simulink library "suspended_payload_lib"  (R2018b)
settings: Solver=VariableStepAuto  StartTime=0.0  StopTime=10.0  RelTol=1e-3
undefined symbols (not defined in the file or in its folder): IC_susp_payload, susp_payload, uav
libraries: axes_transformation_lib x10, flight_parameters_lib x9, unit_conversions_lib x3, vrlib x2, rigidBody_lib x1
settings Model: Creator=jonas  LastModifiedBy=yannic

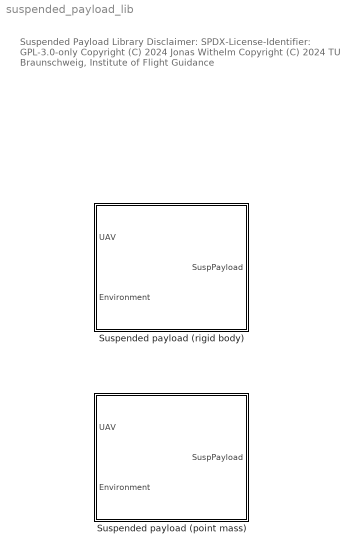
== system suspended_payload_lib ==
  note: Suspended Payload Library
      |
      | Disclaimer:
      | SPDX-License-Identifier: GPL-3.0-only
      |
      | Copyright (C) 2024 Jonas Withelm
      | Copyright (C) 2024 TU Braunschweig, Institute of Flight Guidance
  Suspended payload (point mass) : Subsystem  mask(Suspended payload (point mass)){uav_=uav, susp_payload_=susp_payload, IC_sp_=IC_susp_payload}
      mask prompts: uav_ "uav parameters struct"; susp_payload_ "suspended payload parameters struct"; IC_sp_ "suspended payload initial conditions struct"
      mask help: Point mass suspended payload model (without aerodynamics and joint angle limit)
  Suspended payload (rigid body) : Subsystem  mask(Suspended payload (rigid body)){uav_=uav, susp_payload_=susp_payload, IC_sp_=IC_susp_payload}
      mask prompts: uav_ "uav parameters struct"; susp_payload_ "suspended payload parameters struct"; IC_sp_ "suspended payload initial conditions struct"
      mask help: Rigid body suspended payload model with simple aerodynamics and joint angle limit

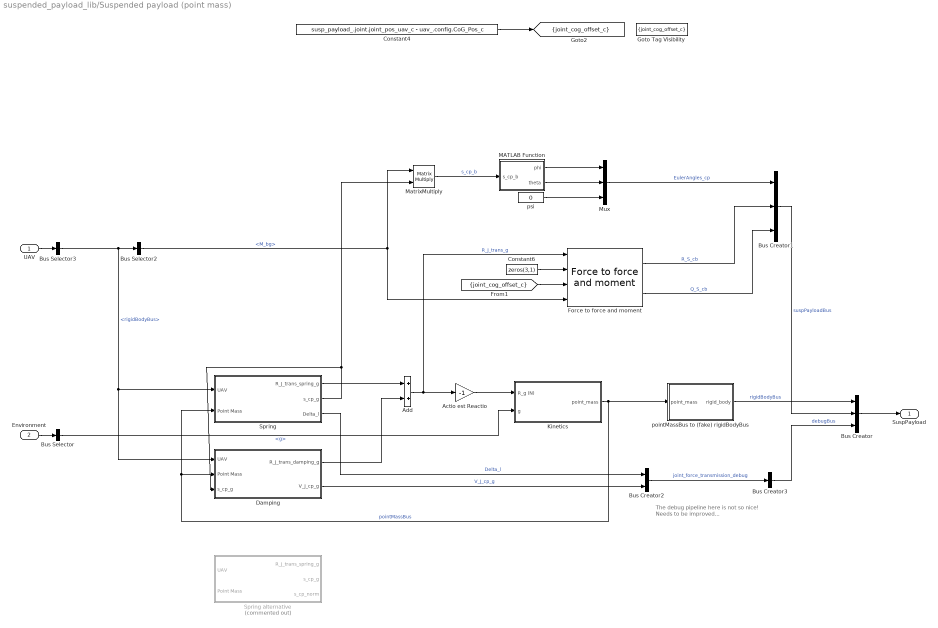
== system suspended_payload_lib/Suspended payload (point mass) ==
  note: The debug pipeline here is not so nice!
      |
      | Needs to be improved...
  UAV : Inport
  Environment : Inport  Port=2
  Actio est Reactio : Gain  Gain=-1
  Add : Sum
  Bus Creator : BusCreator  Inputs=3
  Bus Creator1 : BusCreator  Inputs=3
  Bus Creator2 : BusCreator  Inputs=2
  Bus Creator3 : BusCreator  Inputs=1
  Bus Selector : BusSelector  OutputSignals=g
  Bus Selector2 : BusSelector  OutputSignals=M_bg
  Bus Selector3 : BusSelector  OutputSignals=rigidBodyBus
  Constant4 : Constant  Value=susp_payload_.joint.joint_pos_uav_c - uav_.config.CoG_Pos_c
  Constant6 : Constant  Value=zeros(3,1)
  Damping : Subsystem
  Force to force and moment : axes_transformation_lib/Force to force and moment  SystemSampleTime=-1
      settings: SourceProductName=LADAC
  Goto Tag Visibility : GotoTagVisibility  GotoTag=joint_cog_offset_c
  Kinetics : Subsystem
  MATLAB Function : MATLAB Function  TreatAsAtomicUnit=on
  MatrixMultiply : Product  Multiplication=Matrix(*)
  Mux : Mux  Inputs=3
  Spring : Subsystem
  Spring alternative : Subsystem  Commented=on
  pointMassBus to (fake) rigidBodyBus : Subsystem
  psi : Constant  Value=0
  SuspPayload : Outport
  tag scope: joint_cog_offset_c=scoped
  wires:
  MATLAB Function/1(phi) -> Mux/1
  Constant6/1 -> Force to force and moment/2
  Spring/1(R_J_trans_spring_g) -> Add/1
  [joint_cog_offset_c] -> Force to force and moment/3
  Add/1 -> Force to force and moment/1, Actio est Reactio/1  "R_J_trans_g"
  MATLAB Function/2(theta) -> Mux/2
  MatrixMultiply/1 -> MATLAB Function/1(s_cp_b)  "s_cp_b"
  Bus Creator1/1 -> Bus Creator/2  "suspPayloadBus"
  Force to force and moment/1 -> Bus Creator1/2  "R_S_cb"
  Force to force and moment/2 -> Bus Creator1/3  "Q_S_cb"
  Bus Selector2/1 -> Force to force and moment/4, MatrixMultiply/1  "<M_bg>"
  UAV/1 -> Bus Selector3/1
  Spring/2(s_cp_g) -> MatrixMultiply/2, Damping/3(s_cp_g)
  Damping/1(R_J_trans_damping_g) -> Add/2
  Bus Creator/1 -> SuspPayload/1
  Kinetics/1(point_mass) -> Spring/2(Point Mass), Damping/2(Point Mass), pointMassBus to (fake) rigidBodyBus/1(point_mass)  "pointMassBus"
  pointMassBus to (fake) rigidBodyBus/1(rigid_body) -> Bus Creator/1  "rigidBodyBus"
  Actio est Reactio/1 -> Kinetics/1(R_g (N))
  Spring/3(Delta_l) -> Bus Creator2/1  "Delta_l"
  psi/1 -> Mux/3
  Environment/1 -> Bus Selector/1
  Damping/2(V_J_cp_g) -> Bus Creator2/2  "V_J_cp_g"
  Bus Creator2/1 -> Bus Creator3/1  "joint_force_transmission_debug"
  Bus Creator3/1 -> Bus Creator/3  "debugBus"
  Mux/1 -> Bus Creator1/1  "EulerAngles_cp"
  Bus Selector3/1 -> Spring/1(UAV), Damping/1(UAV), Bus Selector2/1  "<rigidBodyBus>"
  Constant4/1 -> [joint_cog_offset_c]
  Bus Selector/1 -> Kinetics/2(g)  "<g>"

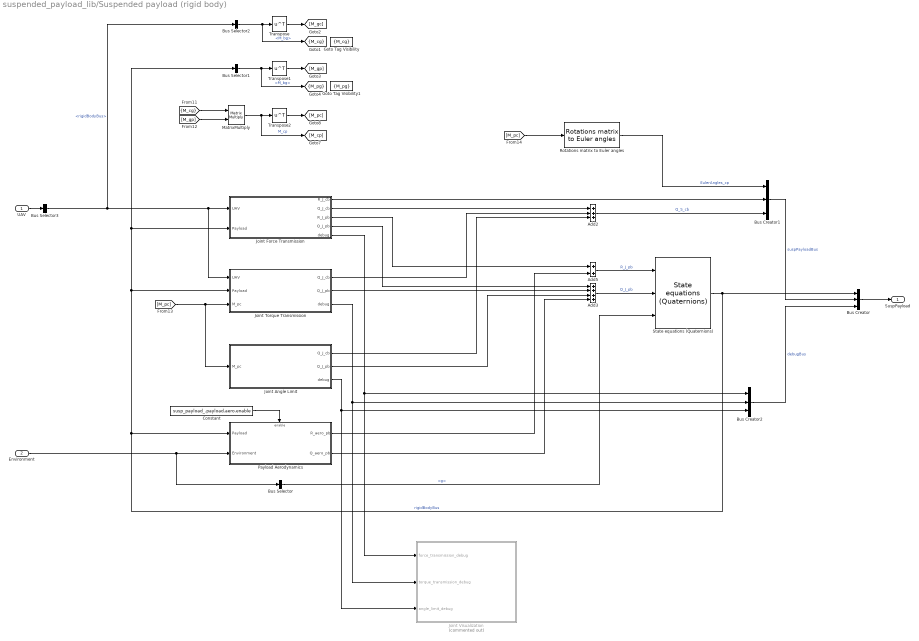
== system suspended_payload_lib/Suspended payload (rigid body) ==
  UAV : Inport
  Environment : Inport  Port=2
  Add2 : Sum  Inputs=+++
  Add3 : Sum  Inputs=++++
  Add5 : Sum
  Bus Creator : BusCreator  Inputs=3
  Bus Creator1 : BusCreator  Inputs=3
  Bus Creator2 : BusCreator  Inputs=3
  Bus Selector : BusSelector  OutputSignals=g
  Bus Selector1 : BusSelector  OutputSignals=M_bg
  Bus Selector2 : BusSelector  OutputSignals=M_bg
  Bus Selector3 : BusSelector  OutputSignals=rigidBodyBus
  Constant : Constant  Value=susp_payload_.payload.aero.enable
  Goto Tag Visibility : GotoTagVisibility  GotoTag=M_cg
  Goto Tag Visibility1 : GotoTagVisibility  GotoTag=M_pg
  Joint Angle Limit : Subsystem
  Joint Force Transmission : Subsystem
  Joint Torque Transmission : Subsystem
  Joint Visualization : Subsystem  Commented=on
  MatrixMultiply : Product  Multiplication=Matrix(*)
  Payload Aerodynamics : Subsystem
  Rotations matrix to Euler angles : axes_transformation_lib/Rotations matrix to Euler angles  SystemSampleTime=-1
      settings: SourceProductName=LADAC
  State equations (Quaternions) : rigidBody_lib/State equations (Quaternions)  m=susp_payload_.body.m  I=susp_payload_.body.I  is_g_checked=on  g=10  omega_Kb_0=IC_sp_.omega_Kb  q_bg_0=IC_sp_.q_bg  V_Kb_0=IC_sp_.V_Kb  s_g_0=IC_sp_.s_g
      settings: SourceProductName=LADAC
  Transpose : Math  Operator=transpose  SaturateOnIntegerOverflow=on
  Transpose1 : Math  Operator=transpose  SaturateOnIntegerOverflow=on
  Transpose2 : Math  Operator=transpose  SaturateOnIntegerOverflow=on
  SuspPayload : Outport
  tag scope: M_cg=scoped, M_pg=scoped
  wires:
  Bus Creator1/1 -> Bus Creator/2  "suspPayloadBus"
  Bus Selector/1 -> State equations (Quaternions)/3  "<g>"
  Add2/1 -> Bus Creator1/3  "Q_S_cb"
  MatrixMultiply/1 -> [M_cp], Transpose2/1  "M_cp"
  [M_gp] -> MatrixMultiply/2
  [M_cg] -> MatrixMultiply/1
  [M_pc] -> Joint Angle Limit/1(M_pc), Joint Torque Transmission/3(M_pc)
  [M_pc] -> Rotations matrix to Euler angles/1
  Transpose2/1 -> [M_pc]
  Add3/1 -> State equations (Quaternions)/2  "Q_J_pb"
  Joint Angle Limit/1(Q_J_cb) -> Add2/3
  Joint Angle Limit/2(Q_J_pb) -> Add3/3
  Joint Torque Transmission/1(Q_J_cb) -> Add2/2
  Joint Torque Transmission/2(Q_J_pb) -> Add3/2
  Environment/1 -> Bus Selector/1, Payload Aerodynamics/2(Environment)
  Add5/1 -> State equations (Quaternions)/1  "R_J_pb"
  Payload Aerodynamics/1(R_aero_pb) -> Add5/2
  Joint Force Transmission/1(R_J_cb) -> Bus Creator1/2
  Joint Force Transmission/2(Q_J_cb) -> Add2/1
  Joint Force Transmission/3(R_J_pb) -> Add5/1
  Joint Force Transmission/4(Q_J_pb) -> Add3/1
  Bus Selector1/1 -> [M_pg], Transpose1/1  "<M_bg>"
  Bus Selector3/1 -> Bus Selector2/1, Joint Torque Transmission/1(UAV), Joint Force Transmission/1(UAV)  "<rigidBodyBus>"
  Bus Selector2/1 -> [M_cg], Transpose/1  "<M_bg>"
  Transpose/1 -> [M_gc]
  Transpose1/1 -> [M_gp]
  Payload Aerodynamics/2(Q_aero_pb) -> Add3/4
  Joint Torque Transmission/3(debug) -> Joint Visualization/2(torque_transmission_debug), Bus Creator2/2
  State equations (Quaternions)/1 -> Bus Creator/1, Bus Selector1/1, Joint Force Transmission/2(Payload), Joint Torque Transmission/2(Payload), Payload Aerodynamics/1(Payload)  "rigidBodyBus"
  Bus Creator/1 -> SuspPayload/1
  Constant/1 -> Payload Aerodynamics/Enable
  Joint Force Transmission/5(debug) -> Joint Visualization/1(force_transmission_debug), Bus Creator2/1
  Bus Creator2/1 -> Bus Creator/3  "debugBus"
  Joint Angle Limit/3(debug) -> Joint Visualization/3(angle_limit_debug), Bus Creator2/3
  Rotations matrix to Euler angles/1 -> Bus Creator1/1  "EulerAngles_cp"
  UAV/1 -> Bus Selector3/1

== system suspended_payload_lib/Suspended payload (point mass)/Damping ==
  UAV : Inport
  Point Mass : Inport  Port=2
  s_cp_g : Inport  Port=3
  Add6 : Sum  Inputs=-+
  Bus Selector : BusSelector  OutputSignals=s_g_dt
  Bus Selector7 : BusSelector  OutputSignals=M_bg,V_Kb,omega_Kb
  Gain : Gain  Gain=susp_payload_.joint.trans_damping
  MatrixMultiply : Product  Multiplication=Matrix(*)
  Transpose : Math  Operator=transpose  SaturateOnIntegerOverflow=on
  Velocity due to rotation2 : axes_transformation_lib/Velocity due to rotation  SystemSampleTime=-1
      settings: SourceProductName=LADAC
  projection of vector a on b : MATLAB Function  TreatAsAtomicUnit=on
  R_J_trans_damping_g : Outport
  V_J_cp_g : Outport  Port=2
  wires:
  MatrixMultiply/1 -> Add6/1  "V_joint_c_g"
  Bus Selector7/3 -> Velocity due to rotation2/2  "<omega_Kb>"
  Velocity due to rotation2/1 -> MatrixMultiply/2
  Bus Selector7/2 -> Velocity due to rotation2/1  "<V_Kb>"
  [joint_cog_offset_c] -> Velocity due to rotation2/3
  Transpose/1 -> MatrixMultiply/1  "M_gc"
  Bus Selector7/1 -> Transpose/1  "<M_bg>"
  UAV/1 -> Bus Selector7/1
  Point Mass/1 -> Bus Selector/1
  Bus Selector/1 -> Add6/2  "<s_g_dt>"
  s_cp_g/1 -> projection of vector a on b/2(b)
  Add6/1 -> projection of vector a on b/1(a)
  projection of vector a on b/1(a_b) -> V_J_cp_g/1, Gain/1
  Gain/1 -> R_J_trans_damping_g/1

== system suspended_payload_lib/Suspended payload (point mass)/Kinetics ==
  R_g (N) : Inport
  g : Inport  Port=2
  Bus Creator : BusCreator  Inputs=3
  Integrator : Integrator  InitialCondition=IC_sp_.V_Kg  ContinuousStateAttributes='velocity_pld'
  Integrator1 : Integrator  InitialCondition=IC_sp_.s_g  ContinuousStateAttributes='position_pld'
  Kinetics : Subsystem
  mass : Constant  Value=susp_payload_.body.m
  point_mass : Outport
  wires:
  Integrator/1 -> Bus Creator/2, Integrator1/1  "s_g_dt"
  R_g (N)/1 -> Kinetics/1(R_g)
  mass/1 -> Kinetics/2(m)
  g/1 -> Kinetics/3(g)
  Kinetics/1(s_Kg_dt2) -> Bus Creator/3, Integrator/1  "s_g_dt2"
  Integrator1/1 -> Bus Creator/1  "s_g"
  Bus Creator/1 -> point_mass/1  "pointMassBus"

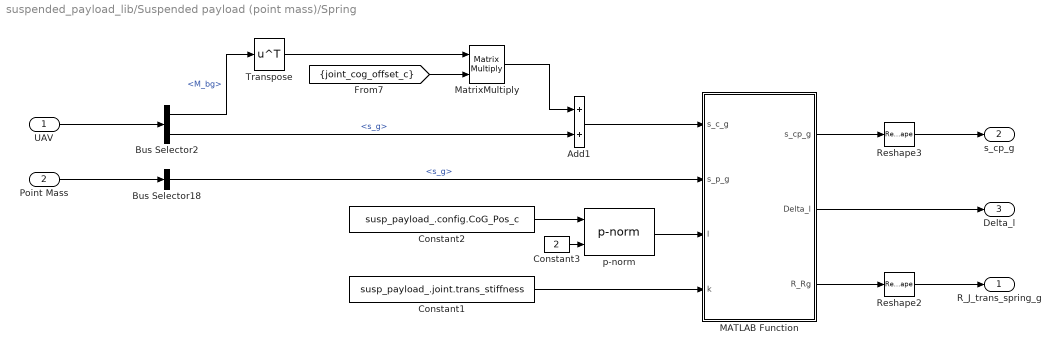
== system suspended_payload_lib/Suspended payload (point mass)/Spring ==
  UAV : Inport
  Point Mass : Inport  Port=2
  Add1 : Sum
  Bus Selector18 : BusSelector  OutputSignals=s_g
  Bus Selector2 : BusSelector  OutputSignals=M_bg,s_g
  Constant1 : Constant  Value=susp_payload_.joint.trans_stiffness
  Constant2 : Constant  Value=susp_payload_.config.CoG_Pos_c
  Constant3 : Constant  Value=2
  MATLAB Function : MATLAB Function  TreatAsAtomicUnit=on
  MatrixMultiply : Product  Multiplication=Matrix(*)
  Reshape2 : Reshape  OutputDimensionality=Column vector (2-D)
  Reshape3 : Reshape  OutputDimensionality=Column vector (2-D)
  Transpose : Math  Operator=transpose  SaturateOnIntegerOverflow=on
  p-norm : flight_parameters_lib/p-norm  SystemSampleTime=-1
      settings: SourceProductName=LADAC
  R_J_trans_spring_g : Outport
  s_cp_g : Outport  Port=2
  Delta_l : Outport  Port=3
  wires:
  Point Mass/1 -> Bus Selector18/1
  MATLAB Function/3(R_Rg) -> Reshape2/1
  Bus Selector18/1 -> MATLAB Function/2(s_p_g)  "<s_g>"
  Reshape2/1 -> R_J_trans_spring_g/1
  Constant1/1 -> MATLAB Function/4(k)
  MATLAB Function/2(Delta_l) -> Delta_l/1
  MATLAB Function/1(s_cp_g) -> Reshape3/1
  Reshape3/1 -> s_cp_g/1
  Transpose/1 -> MatrixMultiply/1
  [joint_cog_offset_c] -> MatrixMultiply/2
  Bus Selector2/2 -> Add1/2  "<s_g>"
  Bus Selector2/1 -> Transpose/1  "<M_bg>"
  MatrixMultiply/1 -> Add1/1
  UAV/1 -> Bus Selector2/1
  Add1/1 -> MATLAB Function/1(s_c_g)
  Constant2/1 -> p-norm/1
  Constant3/1 -> p-norm/2
  p-norm/1 -> MATLAB Function/3(l)

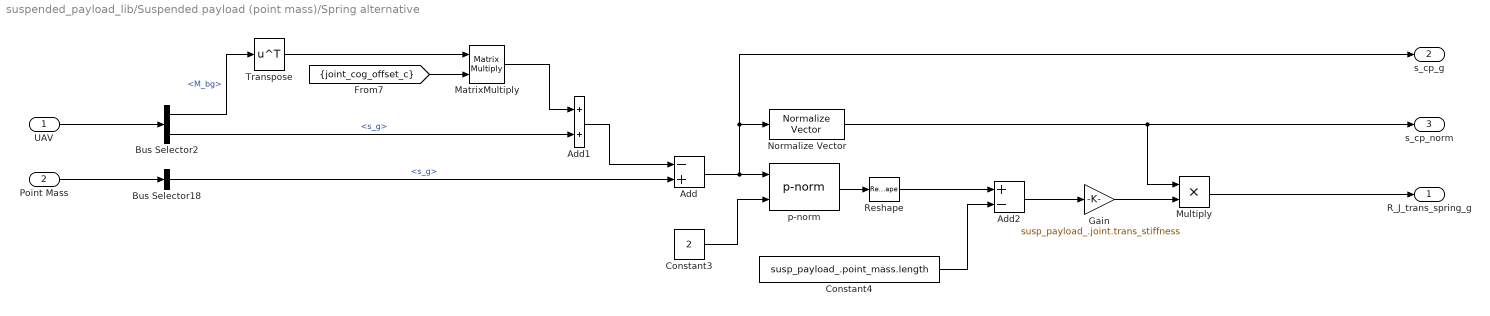
== system suspended_payload_lib/Suspended payload (point mass)/Spring alternative ==
  UAV : Inport
  Point Mass : Inport  Port=2
  Add : Sum  Inputs=-+
  Add1 : Sum
  Add2 : Sum  Inputs=+-
  Bus Selector18 : BusSelector  OutputSignals=s_g
  Bus Selector2 : BusSelector  OutputSignals=M_bg,s_g
  Constant3 : Constant  Value=2
  Constant4 : Constant  Value=susp_payload_.point_mass.length
  Gain : Gain  Gain=susp_payload_.joint.trans_stiffness
  MatrixMultiply : Product  Multiplication=Matrix(*)
  Multiply : Product
  Normalize Vector : vrlib/Utilities/Normalize Vector  maxzero=0
      settings: SourceProductName=Simulink 3D Animation  SourceProductBaseCode=VR
  Reshape : Reshape  OutputDimensionality=Column vector (2-D)
  Transpose : Math  Operator=transpose  SaturateOnIntegerOverflow=on
  p-norm : flight_parameters_lib/p-norm  SystemSampleTime=-1
      settings: SourceProductName=LADAC
  R_J_trans_spring_g : Outport
  s_cp_g : Outport  Port=2
  s_cp_norm : Outport  Port=3
  wires:
  Point Mass/1 -> Bus Selector18/1
  Bus Selector18/1 -> Add/2  "<s_g>"
  Transpose/1 -> MatrixMultiply/1
  [joint_cog_offset_c] -> MatrixMultiply/2
  Bus Selector2/2 -> Add1/2  "<s_g>"
  Bus Selector2/1 -> Transpose/1  "<M_bg>"
  MatrixMultiply/1 -> Add1/1
  UAV/1 -> Bus Selector2/1
  Add1/1 -> Add/1
  Add/1 -> Normalize Vector/1, s_cp_g/1, p-norm/1
  Constant3/1 -> p-norm/2
  p-norm/1 -> Reshape/1
  Constant4/1 -> Add2/2
  Add2/1 -> Gain/1
  Gain/1 -> Multiply/2
  Normalize Vector/1 -> Multiply/1, s_cp_norm/1
  Reshape/1 -> Add2/1
  Multiply/1 -> R_J_trans_spring_g/1

== system suspended_payload_lib/Suspended payload (point mass)/pointMassBus to (fake) rigidBodyBus ==
  point_mass : Inport
  Bus Creator : BusCreator  Inputs=10
  Bus Selector : BusSelector  OutputSignals=s_g,s_g_dt,s_g_dt2
  Constant : Constant  Value=eye(3,3)
  Constant1 : Constant  Value=zeros(3,1)
  Constant2 : Constant  Value=zeros(3,1)
  Constant3 : Constant  Value=zeros(3,1)
  Subsystem : Subsystem
  Subsystem1 : Subsystem
  rigid_body : Outport
  wires:
  Bus Creator/1 -> rigid_body/1
  Bus Selector/1 -> Bus Creator/1  "<s_g>"
  Bus Selector/2 -> Subsystem/1(In1), Subsystem1/1(In1), Bus Creator/2  "<s_g_dt>"
  Bus Selector/3 -> Subsystem/2(In2), Bus Creator/3  "<s_g_dt2>"
  Constant/1 -> Bus Creator/8  "M_bg"
  Constant1/1 -> Bus Creator/9  "omega_Kb"
  Constant2/1 -> Bus Creator/10  "omega_Kb_dt"
  Constant3/1 -> Bus Creator/7  "EulerAngles"
  point_mass/1 -> Bus Selector/1
  Subsystem/1(Out1) -> Bus Creator/5  "V_Kb"
  Subsystem/2(Out2) -> Bus Creator/6  "V_Kb_dt"
  Subsystem1/1(Out1) -> Bus Creator/4  "V_Kg"

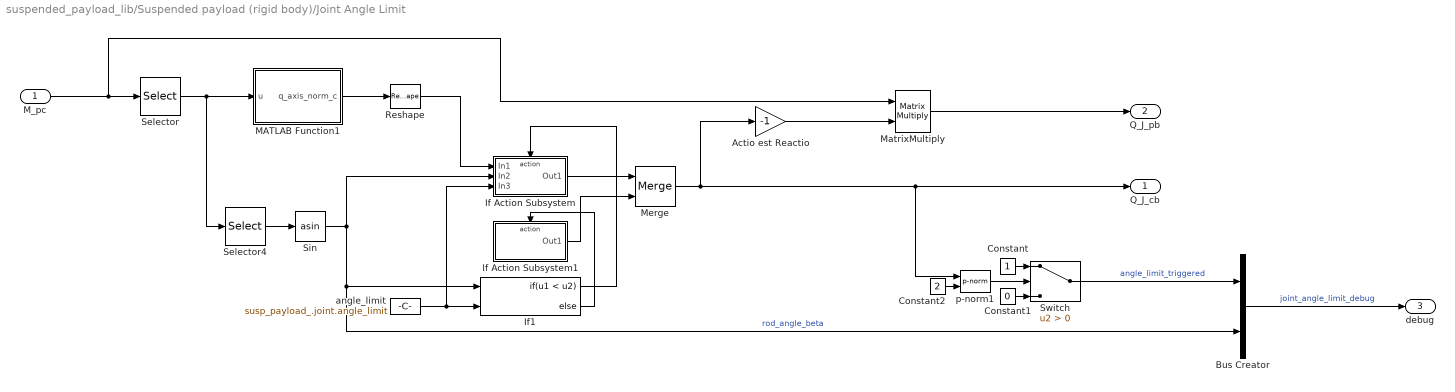
== system suspended_payload_lib/Suspended payload (rigid body)/Joint Angle Limit ==
  M_pc : Inport
  Actio est Reactio : Gain  Gain=-1
  Bus Creator : BusCreator  Inputs=2
  Constant : Constant
  Constant1 : Constant  Value=0
  Constant2 : Constant  Value=2
  If Action Subsystem : Subsystem  TreatAsAtomicUnit=on
  If Action Subsystem1 : Subsystem  TreatAsAtomicUnit=on
  If1 : If  NumInputs=2  IfExpression=u1 < u2
  MATLAB Function1 : MATLAB Function  TreatAsAtomicUnit=on
  MatrixMultiply : Product  Multiplication=Matrix(*)
  Merge : Merge
  Reshape : Reshape  OutputDimensionality=Column vector (2-D)
  Selector : Selector  NumberOfDimensions=2  InputPortWidth=3  IndexOptions=Index vector (dialog),Index vector (dialog)  Indices=[1 2 3],3  OutputSizes=1,1
  Selector4 : Selector  InputPortWidth=3  IndexOptions=Index vector (dialog)  Indices=[3]  OutputSizes=1
  Sin : Trigonometry  Operator=asin
  Switch : Switch  Criteria=u2 > Threshold
  angle_limit : Constant  Value=susp_payload_.joint.angle_limit
  p-norm1 : flight_parameters_lib/p-norm  SystemSampleTime=-1
      settings: SourceProductName=LADAC
  Q_J_cb : Outport
  Q_J_pb : Outport  Port=2
  debug : Outport  Port=3
  wires:
  If1/1 -> If Action Subsystem/Action
  Selector4/1 -> Sin/1
  Actio est Reactio/1 -> MatrixMultiply/2
  MATLAB Function1/1(q_axis_norm_c) -> Reshape/1
  Selector/1 -> MATLAB Function1/1(u), Selector4/1
  Merge/1 -> p-norm1/1, Q_J_cb/1, Actio est Reactio/1
  angle_limit/1 -> If Action Subsystem/3(In3), If1/2
  MatrixMultiply/1 -> Q_J_pb/1
  Reshape/1 -> If Action Subsystem/1(In1)
  M_pc/1 -> MatrixMultiply/1, Selector/1
  Constant/1 -> Switch/1
  Constant1/1 -> Switch/3
  Switch/1 -> Bus Creator/1  "angle_limit_triggered"
  p-norm1/1 -> Switch/2
  Constant2/1 -> p-norm1/2
  If1/2 -> If Action Subsystem1/Action
  If Action Subsystem/1(Out1) -> Merge/1
  If Action Subsystem1/1(Out1) -> Merge/2
  Sin/1 -> If Action Subsystem/2(In2), Bus Creator/2, If1/1  "rod_angle_beta"
  Bus Creator/1 -> debug/1  "joint_angle_limit_debug"

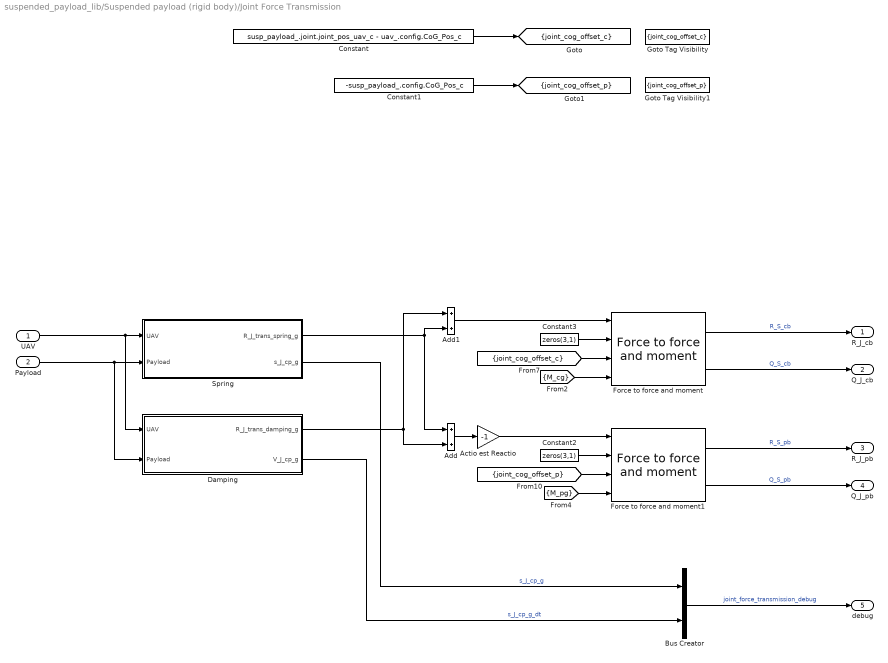
== system suspended_payload_lib/Suspended payload (rigid body)/Joint Force Transmission ==
  UAV : Inport
  Payload : Inport  Port=2
  Actio est Reactio : Gain  Gain=-1
  Add : Sum
  Add1 : Sum
  Bus Creator : BusCreator  Inputs=2
  Constant : Constant  Value=susp_payload_.joint.joint_pos_uav_c - uav_.config.CoG_Pos_c
  Constant1 : Constant  Value=-susp_payload_.config.CoG_Pos_c
  Constant2 : Constant  Value=zeros(3,1)
  Constant3 : Constant  Value=zeros(3,1)
  Damping : Subsystem
  Force to force and moment : axes_transformation_lib/Force to force and moment  SystemSampleTime=-1
      settings: SourceProductName=LADAC
  Force to force and moment1 : axes_transformation_lib/Force to force and moment  SystemSampleTime=-1
      settings: SourceProductName=LADAC
  Goto Tag Visibility : GotoTagVisibility  GotoTag=joint_cog_offset_c
  Goto Tag Visibility1 : GotoTagVisibility  GotoTag=joint_cog_offset_p
  Spring : Subsystem
  R_J_cb : Outport
  Q_J_cb : Outport  Port=2
  R_J_pb : Outport  Port=3
  Q_J_pb : Outport  Port=4
  debug : Outport  Port=5
  tag scope: joint_cog_offset_c=scoped, joint_cog_offset_p=scoped
  wires:
  Constant2/1 -> Force to force and moment1/2
  Force to force and moment/2 -> Q_J_cb/1  "Q_S_cb"
  Force to force and moment1/1 -> R_J_pb/1  "R_S_pb"
  Add1/1 -> Force to force and moment/1
  UAV/1 -> Damping/1(UAV), Spring/1(UAV)
  [joint_cog_offset_p] -> Force to force and moment1/3
  [M_cg] -> Force to force and moment/4
  Force to force and moment/1 -> R_J_cb/1  "R_S_cb"
  Spring/1(R_J_trans_spring_g) -> Add/1, Add1/2
  [joint_cog_offset_c] -> Force to force and moment/3
  Constant3/1 -> Force to force and moment/2
  Force to force and moment1/2 -> Q_J_pb/1  "Q_S_pb"
  [M_pg] -> Force to force and moment1/4
  Add/1 -> Actio est Reactio/1
  Damping/1(R_J_trans_damping_g) -> Add1/1, Add/2
  Payload/1 -> Damping/2(Payload), Spring/2(Payload)
  Damping/2(V_J_cp_g) -> Bus Creator/2  "s_J_cp_g_dt"
  Spring/2(s_J_cp_g) -> Bus Creator/1  "s_J_cp_g"
  Actio est Reactio/1 -> Force to force and moment1/1
  Bus Creator/1 -> debug/1  "joint_force_transmission_debug"
  Constant/1 -> [joint_cog_offset_c]
  Constant1/1 -> [joint_cog_offset_p]

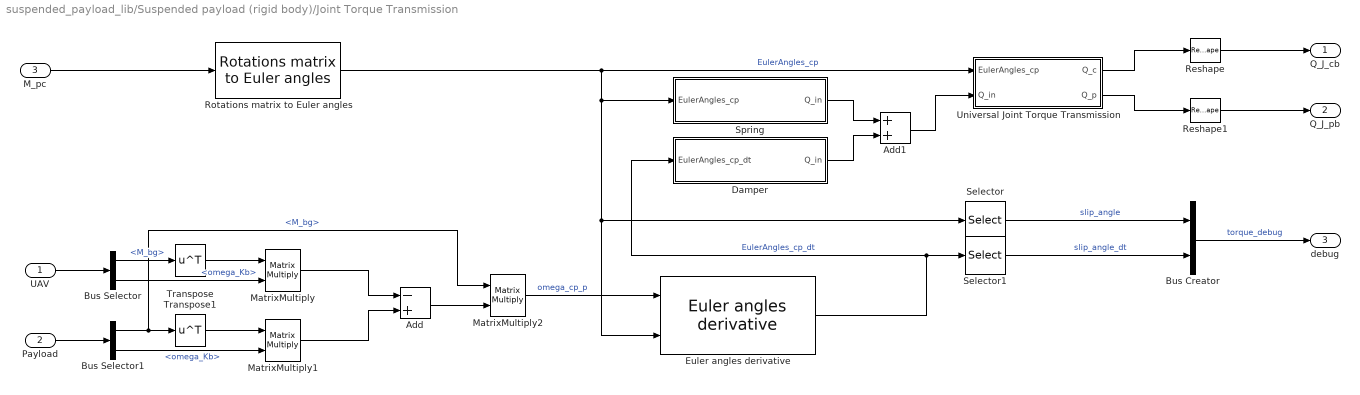
== system suspended_payload_lib/Suspended payload (rigid body)/Joint Torque Transmission ==
  UAV : Inport
  Payload : Inport  Port=2
  M_pc : Inport  Port=3
  Add : Sum  Inputs=-+
  Add1 : Sum
  Bus Creator : BusCreator  Inputs=2
  Bus Selector : BusSelector  OutputSignals=M_bg,omega_Kb
  Bus Selector1 : BusSelector  OutputSignals=M_bg,omega_Kb
  Damper : Subsystem
  Euler angles derivative : flight_parameters_lib/Euler angles derivative  SystemSampleTime=-1
      settings: SourceProductName=LADAC
  MatrixMultiply : Product  Multiplication=Matrix(*)
  MatrixMultiply1 : Product  Multiplication=Matrix(*)
  MatrixMultiply2 : Product  Multiplication=Matrix(*)
  Reshape : Reshape  OutputDimensionality=Column vector (2-D)
  Reshape1 : Reshape  OutputDimensionality=Column vector (2-D)
  Rotations matrix to Euler angles : axes_transformation_lib/Rotations matrix to Euler angles  SystemSampleTime=-1
      settings: SourceProductName=LADAC
  Selector : Selector  InputPortWidth=3  IndexOptions=Index vector (dialog)  Indices=[3]  OutputSizes=1
  Selector1 : Selector  InputPortWidth=3  IndexOptions=Index vector (dialog)  Indices=[3]  OutputSizes=1
  Spring : Subsystem
  Transpose : Math  Operator=transpose  SaturateOnIntegerOverflow=on
  Transpose1 : Math  Operator=transpose  SaturateOnIntegerOverflow=on
  Universal Joint Torque Transmission : MATLAB Function  TreatAsAtomicUnit=on
  Q_J_cb : Outport
  Q_J_pb : Outport  Port=2
  debug : Outport  Port=3
  wires:
  Reshape1/1 -> Q_J_pb/1
  M_pc/1 -> Rotations matrix to Euler angles/1
  Universal Joint Torque Transmission/1(Q_c) -> Reshape/1
  Universal Joint Torque Transmission/2(Q_p) -> Reshape1/1
  Reshape/1 -> Q_J_cb/1
  Rotations matrix to Euler angles/1 -> Spring/1(EulerAngles_cp), Euler angles derivative/2, Selector/1, Universal Joint Torque Transmission/1(EulerAngles_cp)  "EulerAngles_cp"
  Selector/1 -> Bus Creator/1  "slip_angle"
  UAV/1 -> Bus Selector/1
  Payload/1 -> Bus Selector1/1
  Bus Selector/1 -> Transpose/1  "<M_bg>"
  Transpose/1 -> MatrixMultiply/1
  Bus Selector/2 -> MatrixMultiply/2  "<omega_Kb>"
  Transpose1/1 -> MatrixMultiply1/1
  Bus Selector1/2 -> MatrixMultiply1/2  "<omega_Kb>"
  Bus Selector1/1 -> MatrixMultiply2/1, Transpose1/1  "<M_bg>"
  MatrixMultiply/1 -> Add/1
  MatrixMultiply1/1 -> Add/2
  Add/1 -> MatrixMultiply2/2
  MatrixMultiply2/1 -> Euler angles derivative/1  "omega_cp_p"
  Bus Creator/1 -> debug/1  "torque_debug"
  Selector1/1 -> Bus Creator/2  "slip_angle_dt"
  Euler angles derivative/1 -> Damper/1(EulerAngles_cp_dt), Selector1/1  "EulerAngles_cp_dt"
  Spring/1(Q_in) -> Add1/1
  Damper/1(Q_in) -> Add1/2
  Add1/1 -> Universal Joint Torque Transmission/2(Q_in)

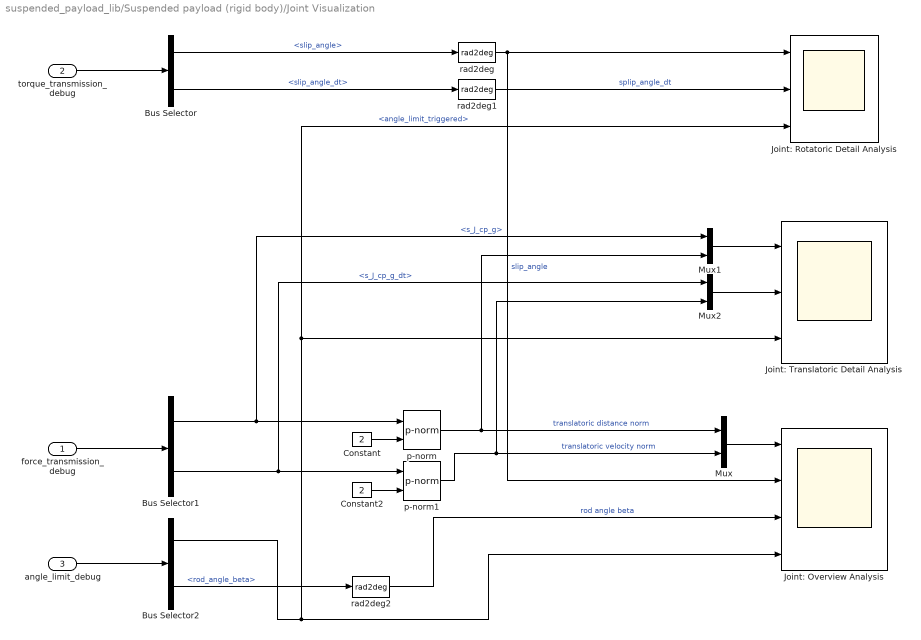
== system suspended_payload_lib/Suspended payload (rigid body)/Joint Visualization ==
  force_transmission_debug : Inport
  torque_transmission_debug : Inport  Port=2
  angle_limit_debug : Inport  Port=3
  Bus Selector : BusSelector  OutputSignals=slip_angle,slip_angle_dt
  Bus Selector1 : BusSelector  OutputSignals=s_J_cp_g,s_J_cp_g_dt
  Bus Selector2 : BusSelector  OutputSignals=angle_limit_triggered,rod_angle_beta
  Constant : Constant  Value=2
  Constant2 : Constant  Value=2
  Joint: Overview Analysis : Scope  NumInputPorts=4
  Joint: Rotatoric Detail Analysis : Scope  NumInputPorts=3
  Joint: Translatoric Detail Analysis : Scope  NumInputPorts=3
  Mux : Mux  Inputs=2
  Mux1 : Mux  Inputs=2
  Mux2 : Mux  Inputs=2
  p-norm : flight_parameters_lib/p-norm  SystemSampleTime=-1
      settings: SourceProductName=LADAC
  p-norm1 : flight_parameters_lib/p-norm  SystemSampleTime=-1
      settings: SourceProductName=LADAC
  rad2deg : unit_conversions_lib/rad2deg
      settings: SourceProductName=LADAC
  rad2deg1 : unit_conversions_lib/rad2deg
      settings: SourceProductName=LADAC
  rad2deg2 : unit_conversions_lib/rad2deg
      settings: SourceProductName=LADAC
  wires:
  Mux/1 -> Joint: Overview Analysis/1
  Bus Selector2/1 -> Joint: Overview Analysis/4, Joint: Rotatoric Detail Analysis/3, Joint: Translatoric Detail Analysis/3  "<angle_limit_triggered>"
  Constant/1 -> p-norm/2
  Constant2/1 -> p-norm1/2
  p-norm/1 -> Mux1/2, Mux/1  "translatoric distance norm"
  p-norm1/1 -> Mux2/2, Mux/2  "translatoric velocity norm"
  torque_transmission_debug/1 -> Bus Selector/1
  rad2deg2/1 -> Joint: Overview Analysis/3  "rod angle beta"
  Mux1/1 -> Joint: Translatoric Detail Analysis/1
  Mux2/1 -> Joint: Translatoric Detail Analysis/2
  Bus Selector/1 -> rad2deg/1  "<slip_angle>"
  Bus Selector/2 -> rad2deg1/1  "<slip_angle_dt>"
  rad2deg/1 -> Joint: Overview Analysis/2, Joint: Rotatoric Detail Analysis/1  "slip_angle"
  rad2deg1/1 -> Joint: Rotatoric Detail Analysis/2  "splip_angle_dt"
  force_transmission_debug/1 -> Bus Selector1/1
  angle_limit_debug/1 -> Bus Selector2/1
  Bus Selector1/1 -> Mux1/1, p-norm/1  "<s_J_cp_g>"
  Bus Selector1/2 -> Mux2/1, p-norm1/1  "<s_J_cp_g_dt>"
  Bus Selector2/2 -> rad2deg2/1  "<rod_angle_beta>"

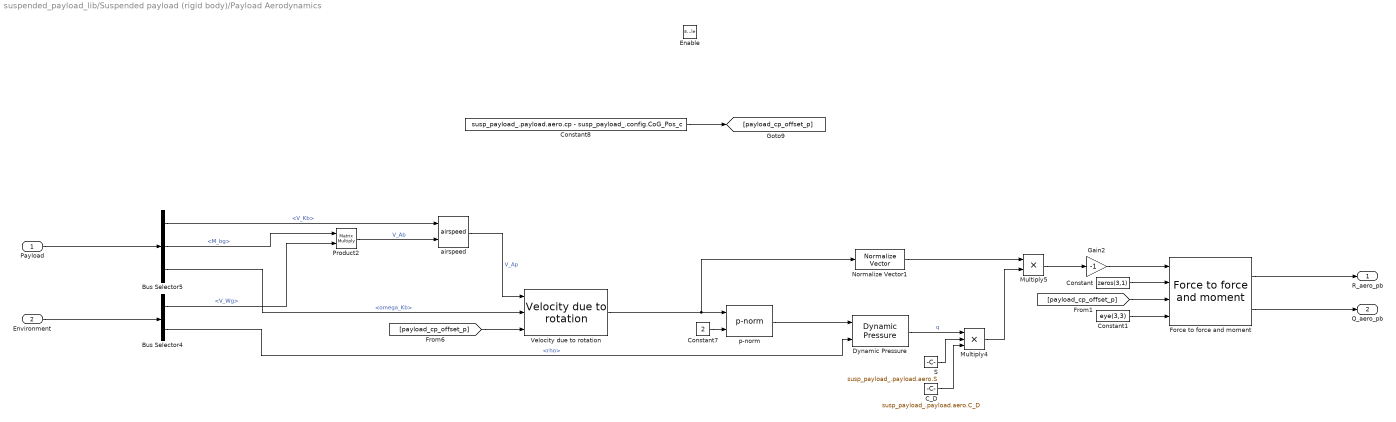
== system suspended_payload_lib/Suspended payload (rigid body)/Payload Aerodynamics ==
  Payload : Inport
  Environment : Inport  Port=2
  Enable : EnablePort
  Bus Selector4 : BusSelector  OutputSignals=wind.V_Wg,atmosphere.rho
  Bus Selector5 : BusSelector  OutputSignals=V_Kb,M_bg,omega_Kb
  C_D : Constant  Value=susp_payload_.payload.aero.C_D
  Constant : Constant  Value=zeros(3,1)
  Constant1 : Constant  Value=eye(3,3)
  Constant7 : Constant  Value=2
  Constant8 : Constant  Value=susp_payload_.payload.aero.cp - susp_payload_.config.CoG_Pos_c
  Dynamic Pressure : flight_parameters_lib/Dynamic Pressure
      settings: SourceProductName=LADAC
  Force to force and moment : axes_transformation_lib/Force to force and moment  SystemSampleTime=-1
      settings: SourceProductName=LADAC
  Gain2 : Gain  Gain=-1
  Multiply4 : Product  Inputs=3
  Multiply5 : Product
  Normalize Vector1 : vrlib/Utilities/Normalize Vector  maxzero=0
      settings: SourceProductName=Simulink 3D Animation  SourceProductBaseCode=VR
  Product2 : Product  Multiplication=Matrix(*)
  S : Constant  Value=susp_payload_.payload.aero.S
  Velocity due to rotation : axes_transformation_lib/Velocity due to rotation  SystemSampleTime=-1
      settings: SourceProductName=LADAC
  airspeed : flight_parameters_lib/airspeed
      settings: SourceProductName=LADAC
  p-norm : flight_parameters_lib/p-norm  SystemSampleTime=-1
      settings: SourceProductName=LADAC
  R_aero_pb : Outport
  Q_aero_pb : Outport  Port=2
  wires:
  Constant7/1 -> p-norm/2
  Bus Selector4/2 -> Dynamic Pressure/2  "<rho>"
  C_D/1 -> Multiply4/3
  p-norm/1 -> Dynamic Pressure/1
  [payload_cp_offset_p] -> Velocity due to rotation/3
  S/1 -> Multiply4/2
  airspeed/1 -> Velocity due to rotation/1  "V_Ap"
  Bus Selector5/2 -> Product2/1  "<M_bg>"
  Product2/1 -> airspeed/2  "V_Ab"
  Bus Selector4/1 -> Product2/2  "<V_Wg>"
  Environment/1 -> Bus Selector4/1
  Velocity due to rotation/1 -> p-norm/1, Normalize Vector1/1
  Payload/1 -> Bus Selector5/1
  Multiply4/1 -> Multiply5/2
  Multiply5/1 -> Gain2/1
  Bus Selector5/1 -> airspeed/1  "<V_Kb>"
  Gain2/1 -> Force to force and moment/1
  Dynamic Pressure/1 -> Multiply4/1  "q"
  Bus Selector5/3 -> Velocity due to rotation/2  "<omega_Kb>"
  Normalize Vector1/1 -> Multiply5/1
  Constant8/1 -> [payload_cp_offset_p]
  Constant/1 -> Force to force and moment/2
  Constant1/1 -> Force to force and moment/4
  [payload_cp_offset_p] -> Force to force and moment/3
  Force to force and moment/1 -> R_aero_pb/1
  Force to force and moment/2 -> Q_aero_pb/1

== system suspended_payload_lib/Suspended payload (point mass)/Kinetics/Kinetics ==
  R_g : Inport
  m : Inport  Port=2
  g : Inport  Port=3
  MATLAB Function : MATLAB Function  TreatAsAtomicUnit=on
  Reshape : Reshape  OutputDimensionality=Column vector (2-D)
  Reshape4 : Reshape  OutputDimensionality=Column vector (2-D)
  s_Kg_dt2 : Outport
  wires:
  Reshape4/1 -> s_Kg_dt2/1
  g/1 -> MATLAB Function/3(g)
  R_g/1 -> Reshape/1
  MATLAB Function/1(s_Kg_dt2) -> Reshape4/1
  m/1 -> MATLAB Function/2(m)
  Reshape/1 -> MATLAB Function/1(R_g)

== system suspended_payload_lib/Suspended payload (point mass)/pointMassBus to (fake) rigidBodyBus/Subsystem ==
  In1 : Inport
  In2 : Inport  Port=2
  Out1 : Outport
  Out2 : Outport  Port=2
  wires:
  In1/1 -> Out1/1
  In2/1 -> Out2/1

== system suspended_payload_lib/Suspended payload (point mass)/pointMassBus to (fake) rigidBodyBus/Subsystem1 ==
  In1 : Inport
  Out1 : Outport
  wires:
  In1/1 -> Out1/1

== system suspended_payload_lib/Suspended payload (rigid body)/Joint Angle Limit/If Action Subsystem ==
  In1 : Inport
  In2 : Inport  Port=2
  In3 : Inport  Port=3
  Action Port : ActionPort  InitializeStates=reset
  Add : Sum  Inputs=+-
  Gain : Gain  Gain=susp_payload_.joint.angle_limit_stiffness
  Multiply : Product
  Out1 : Outport
  wires:
  In1/1 -> Multiply/1
  In2/1 -> Add/1
  In3/1 -> Add/2
  Add/1 -> Gain/1
  Multiply/1 -> Out1/1
  Gain/1 -> Multiply/2

== system suspended_payload_lib/Suspended payload (rigid body)/Joint Angle Limit/If Action Subsystem1 ==
  Action Port : ActionPort
  Constant : Constant  Value=[0;0;0]  VectorParams1D=off
  Out1 : Outport
  wires:
  Constant/1 -> Out1/1

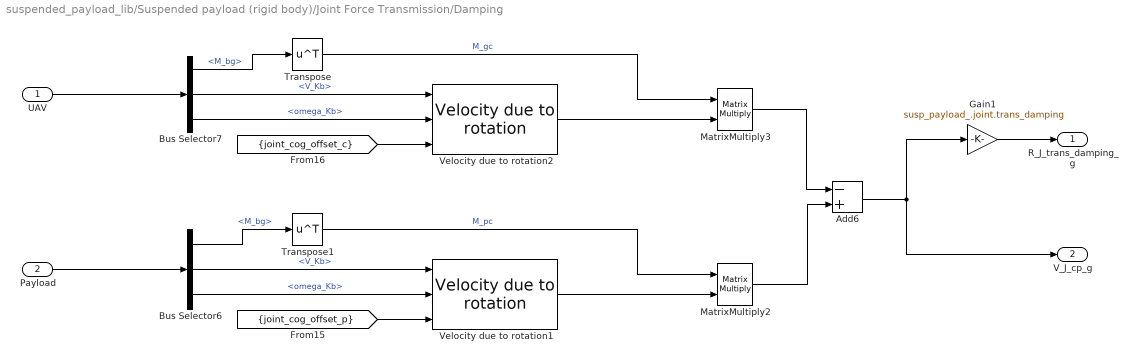
== system suspended_payload_lib/Suspended payload (rigid body)/Joint Force Transmission/Damping ==
  UAV : Inport
  Payload : Inport  Port=2
  Add6 : Sum  Inputs=-+
  Bus Selector6 : BusSelector  OutputSignals=M_bg,V_Kb,omega_Kb
  Bus Selector7 : BusSelector  OutputSignals=M_bg,V_Kb,omega_Kb
  Gain1 : Gain  Gain=susp_payload_.joint.trans_damping
  MatrixMultiply2 : Product  Multiplication=Matrix(*)
  MatrixMultiply3 : Product  Multiplication=Matrix(*)
  Transpose : Math  Operator=transpose  SaturateOnIntegerOverflow=on
  Transpose1 : Math  Operator=transpose  SaturateOnIntegerOverflow=on
  Velocity due to rotation1 : axes_transformation_lib/Velocity due to rotation  SystemSampleTime=-1
      settings: SourceProductName=LADAC
  Velocity due to rotation2 : axes_transformation_lib/Velocity due to rotation  SystemSampleTime=-1
      settings: SourceProductName=LADAC
  R_J_trans_damping_g : Outport
  V_J_cp_g : Outport  Port=2
  wires:
  Velocity due to rotation1/1 -> MatrixMultiply2/2
  Bus Selector6/3 -> Velocity due to rotation1/2  "<omega_Kb>"
  [joint_cog_offset_p] -> Velocity due to rotation1/3
  MatrixMultiply3/1 -> Add6/1
  [joint_cog_offset_c] -> Velocity due to rotation2/3
  Bus Selector7/2 -> Velocity due to rotation2/1  "<V_Kb>"
  Gain1/1 -> R_J_trans_damping_g/1
  Add6/1 -> V_J_cp_g/1, Gain1/1
  Payload/1 -> Bus Selector6/1
  MatrixMultiply2/1 -> Add6/2
  Transpose1/1 -> MatrixMultiply2/1  "M_pc"
  UAV/1 -> Bus Selector7/1
  Bus Selector6/2 -> Velocity due to rotation1/1  "<V_Kb>"
  Velocity due to rotation2/1 -> MatrixMultiply3/2
  Bus Selector7/3 -> Velocity due to rotation2/2  "<omega_Kb>"
  Bus Selector7/1 -> Transpose/1  "<M_bg>"
  Transpose/1 -> MatrixMultiply3/1  "M_gc"
  Bus Selector6/1 -> Transpose1/1  "<M_bg>"

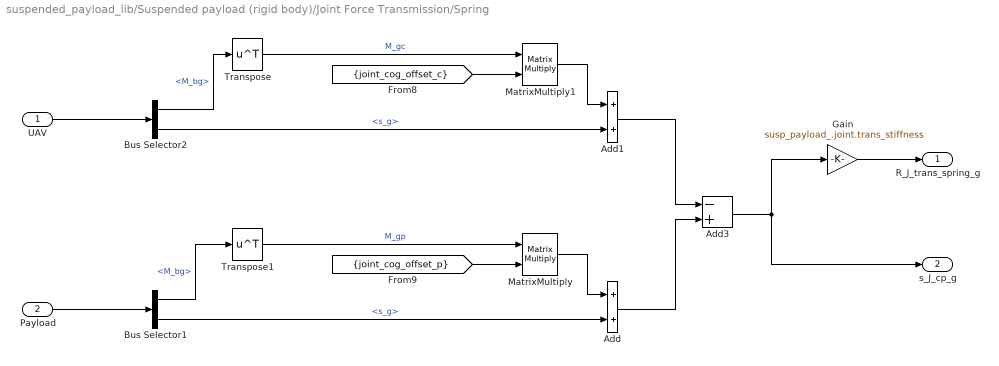
== system suspended_payload_lib/Suspended payload (rigid body)/Joint Force Transmission/Spring ==
  UAV : Inport
  Payload : Inport  Port=2
  Add : Sum
  Add1 : Sum
  Add3 : Sum  Inputs=-+
  Bus Selector1 : BusSelector  OutputSignals=M_bg,s_g
  Bus Selector2 : BusSelector  OutputSignals=M_bg,s_g
  Gain : Gain  Gain=susp_payload_.joint.trans_stiffness
  MatrixMultiply : Product  Multiplication=Matrix(*)
  MatrixMultiply1 : Product  Multiplication=Matrix(*)
  Transpose : Math  Operator=transpose  SaturateOnIntegerOverflow=on
  Transpose1 : Math  Operator=transpose  SaturateOnIntegerOverflow=on
  R_J_trans_spring_g : Outport
  s_J_cp_g : Outport  Port=2
  wires:
  [joint_cog_offset_c] -> MatrixMultiply1/2
  Transpose1/1 -> MatrixMultiply/1  "M_gp"
  Add/1 -> Add3/2
  Bus Selector2/1 -> Transpose/1  "<M_bg>"
  Add1/1 -> Add3/1
  Transpose/1 -> MatrixMultiply1/1  "M_gc"
  Gain/1 -> R_J_trans_spring_g/1
  MatrixMultiply1/1 -> Add1/1
  UAV/1 -> Bus Selector2/1
  [joint_cog_offset_p] -> MatrixMultiply/2
  Bus Selector2/2 -> Add1/2  "<s_g>"
  MatrixMultiply/1 -> Add/1
  Payload/1 -> Bus Selector1/1
  Bus Selector1/1 -> Transpose1/1  "<M_bg>"
  Bus Selector1/2 -> Add/2  "<s_g>"
  Add3/1 -> s_J_cp_g/1, Gain/1

== system suspended_payload_lib/Suspended payload (rigid body)/Joint Torque Transmission/Damper ==
  EulerAngles_cp_dt : Inport
  Constant : Constant  Value=- susp_payload_.joint.rot_damping
  Multiply : Product
  Selector : Selector  InputPortWidth=3  IndexOptions=Index vector (dialog)  Indices=[3]  OutputSizes=1
  Q_in : Outport
  wires:
  Selector/1 -> Multiply/2  "slip_angle_dt"
  Multiply/1 -> Q_in/1
  EulerAngles_cp_dt/1 -> Selector/1
  Constant/1 -> Multiply/1

== system suspended_payload_lib/Suspended payload (rigid body)/Joint Torque Transmission/Spring ==
  EulerAngles_cp : Inport
  Constant : Constant  Value=- susp_payload_.joint.rot_stiffness
  Multiply : Product
  Selector : Selector  InputPortWidth=3  IndexOptions=Index vector (dialog)  Indices=[3]  OutputSizes=1
  Q_in : Outport
  wires:
  EulerAngles_cp/1 -> Selector/1
  Constant/1 -> Multiply/1
  Selector/1 -> Multiply/2  "slip angle"
  Multiply/1 -> Q_in/1

== matlab function suspended_payload_lib/Suspended payload (point mass)/Damping/projection of vector a on b ==
  data: a input; a_b output; b input
function a_b = fcn(a, b)

    % Projection of vector a on vector b:
    a_b = dot(a, b)/dot(b, b) * b;
    
end

== matlab function suspended_payload_lib/Suspended payload (point mass)/Kinetics/Kinetics/MATLAB Function ==
  data: R_g input; s_Kg_dt2 output; m input; g input
function s_Kg_dt2 = fcn(R_g, m, g)
    
    s_Kg_dt2 = R_g/m + [0; 0; g];

end

== matlab function suspended_payload_lib/Suspended payload (point mass)/MATLAB Function ==
  data: s_cp_b input; phi output; theta output
function [phi, theta] = fcn(s_cp_b)
    
    s_cp_norm = norm(s_cp_b);
    
    theta = atan2(s_cp_b(1), s_cp_b(3));
    % Singularity for x=(s_cp_b(1)=z=s_cp_b(3)=0
    
    phi = -asin(s_cp_b(2)/s_cp_norm);
    
end

== matlab function suspended_payload_lib/Suspended payload (rigid body)/Joint Torque Transmission/Universal Joint Torque Transmission ==
  data: EulerAngles_cp input; Q_c output; Q_in input; Q_p output
function [Q_c, Q_p] = fcn(EulerAngles_cp, Q_in)
    
    phi_k = EulerAngles_cp(1);
    theta_k = EulerAngles_cp(2);
    
    
    
    Q_cross_shaft = Q_in / cos(theta_k);
%     Q_x_c = -tan(theta) * Q_in; % Hier würde ich sagen das Vorzeichen ist falsch!
    Q_x_c = tan(theta_k) * Q_in; % So müsste es richtig sein...
    
    Q_y_p = Q_cross_shaft * sin(phi_k);
    Q_z_p = Q_cross_shaft * cos(phi_k);
    
    % Torque out
    Q_c = -[Q_x_c; 0; Q_in];    % Actio est Reactio
    Q_p = [0; Q_y_p; Q_z_p];

end

== matlab function suspended_payload_lib/Suspended payload (rigid body)/Joint Angle Limit/MATLAB Function1 ==
  data: u input; q_axis_norm_c output
function q_axis_norm_c = fcn(u)
    
    s_1 = [0;0;1];
    s_2 = u;
    
    q_axis_c = cross(s_1, s_2);
    
    q_axis_norm_c = 1/norm(q_axis_c) * q_axis_c;
    
end

== matlab function suspended_payload_lib/Suspended payload (point mass)/Spring/MATLAB Function ==
  data: s_cp_g output; Delta_l output; s_c_g input; R_Rg output; s_p_g input; l input; k input
function [s_cp_g, Delta_l, R_Rg] = fcn(s_c_g, s_p_g, l, k)
    
    s_cp_g = s_p_g - s_c_g;
    
    s_cp_norm = vecnorm(s_cp_g);
    s_cp_g_unit = s_cp_g/s_cp_norm;
    
    Delta_l = s_cp_norm - l;
    
    rod_force = Delta_l * k;
    
    R_Rg = s_cp_g_unit * rod_force;

end
